simulink model "Koudruped_simcape"  (R2025b)
settings: Solver=VariableStepAuto  StartTime=0.0  StopTime=30  RelTol=1e-2
undefined symbols (not defined in the file or in its folder): fractalcoef, smiData, X, Y, Z
libraries: sm_lib x589, nesl_utility x93, slpidlib x5, mspsensorlib x4, simulink_extras x4, mspfiltlib x3, simulink x2
(part 16 of 16)

== matlab function Koudruped_simcape/Right Back Step2/MATLAB Function1 ==
  data: t input; pos output; phase_offset input; H_hedef input
function pos = fcn(t, phase_offset, H_hedef)
    pos = zeros(3,1); 
    
    % --- PARAMETRELER (Senin Orijinal Değerlerin) ---
    T_kalkis = 2.0;      
    T_bekleme = 1.0;     
    T_periyot = 1.0;     
    Duty_Factor = 0.5;   
    
    L_adim = 80;         
    H_adim = 30;         
    H_baslangic = -50;   
    Y_offset = 60;       
    
    % --- DURUM MAKİNESİ ---
    if t < T_kalkis
        z = H_baslangic + (H_hedef - H_baslangic) * (t / T_kalkis);
        x = 0;
        pos = [x; Y_offset; z];
        
    elseif t < (T_kalkis + T_bekleme)
        z = H_hedef;
        x = 0;
        pos = [x; Y_offset; z];
        
    else
        t_yurume = t - (T_kalkis + T_bekleme);
        
        T_fade = 2.0; 
        k_amp = min(t_yurume / T_fade, 1.0); 
        
        L_aktif = L_adim * k_amp;
        H_aktif = H_adim * k_amp;
        
        t_norm = mod((t_yurume / T_periyot) + phase_offset, 1.0);
        
        if t_norm < Duty_Factor
            % --- SWING PHASE (HAVADA İLERİ ATILMA) ---
            t_swing = t_norm / Duty_Factor; 
            
            x = (L_aktif/2) - L_aktif * (t_swing - sin(2*pi*t_swing)/(2*pi));
            z = H_hedef + H_aktif * sin(pi * t_swing); 
        else
            % --- STANCE PHASE (YERDE İTME) ---
            t_stance = (t_norm - Duty_Factor) / (1 - Duty_Factor);
            
            x_start = -(L_aktif/2);
            x_end = (L_aktif/2);
            x = x_start + (x_end - x_start) * ((1 - cos(pi * t_stance)) / 2);
            z = H_hedef;
        end
        
        pos = [x; Y_offset; z];
    end
end

== matlab function Koudruped_simcape/Right Back Step2/MATLAB Function2 ==
  data: pos input; angles output
function angles = inverse(pos)
    x = pos(1); y = pos(2); z = pos(3);
    
    % --- PARAMETRELER (Senin değerlerin) ---
    L1 = 44.41; a1 = 24.51; L2 = 100; L3 = 100;
    
    % --- 1. OMUZ (ROLL) ---
    theta1_rad = atan2(y, -z) - atan2(L1, sqrt(y^2 + z^2 - L1^2));

    % --- 2. YARDIMCI KOORDİNATLAR ---
    % Bacak düzlemindeki izdüşüm
    r = sqrt(y^2 + z^2 - L1^2) - a1;
    % Yeni düzlemde hedef noktası (x, r)
    dist_sq = x^2 + r^2;
    dist = sqrt(dist_sq);

    % --- 3. DİZ (KNEE) ---
    cos_phi = (L2^2 + L3^2 - dist_sq) / (2 * L2 * L3);
    cos_phi = min(max(cos_phi, -1), 1); % Sayısal koruma
    phi = acos(cos_phi);
    theta3_rad = (pi - phi); 

    % --- 4. KALÇA (PITCH) ---
    alpha = atan2(x, r);
cos_beta = (L2^2 + dist_sq - L3^2) / (2 * L2 * dist);
cos_beta = min(max(cos_beta, -1), 1);  % Sayısal koruma
beta = acos(cos_beta);
    theta2_rad = alpha + beta;

    % RAD -> DEG
    angles = [theta1_rad; theta2_rad; theta3_rad] * (180/pi);
end

== matlab function Koudruped_simcape/Right Front Step2/MATLAB Function12 ==
  data: t input; pos output; phase_offset input; H_hedef input
function pos = fcn(t, phase_offset, H_hedef)
    pos = zeros(3,1); 
    
    % --- PARAMETRELER  ---
    T_kalkis = 2.0;      
    T_bekleme = 1.0;     
    T_periyot = 1.0;     
    Duty_Factor = 0.5;   
    
    L_adim = 80;         
    H_adim = 30;         
    H_baslangic = -50;   
    Y_offset = 60;       
    
    % --- DURUM MAKİNESİ ---
    if t < T_kalkis
        z = H_baslangic + (H_hedef - H_baslangic) * (t / T_kalkis);
        x = 0;
        pos = [x; Y_offset; z];
        
    elseif t < (T_kalkis + T_bekleme)
        z = H_hedef;
        x = 0;
        pos = [x; Y_offset; z];
        
    else
        t_yurume = t - (T_kalkis + T_bekleme);
        
        T_fade = 2.0; 
        k_amp = min(t_yurume / T_fade, 1.0); 
        
        L_aktif = L_adim * k_amp;
        H_aktif = H_adim * k_amp;
        
        t_norm = mod((t_yurume / T_periyot) + phase_offset, 1.0);
        
        if t_norm < Duty_Factor
            % --- SWING PHASE (HAVADA İLERİ ATILMA) ---
            t_swing = t_norm / Duty_Factor; 
            
            x = (L_aktif/2) - L_aktif * (t_swing - sin(2*pi*t_swing)/(2*pi));
            z = H_hedef + H_aktif * sin(pi * t_swing); 
        else
            % --- STANCE PHASE (YERDE İTME) ---
            t_stance = (t_norm - Duty_Factor) / (1 - Duty_Factor);
            
            x_start = -(L_aktif/2);
            x_end = (L_aktif/2);
            x = x_start + (x_end - x_start) * ((1 - cos(pi * t_stance)) / 2);
            z = H_hedef;
        end
        
        pos = [x; Y_offset; z];
    end
end

== matlab function Koudruped_simcape/Right Front Step2/MATLAB Function13 ==
  data: pos input; angles output
function angles = inverse(pos)
    x = pos(1); y = pos(2); z = pos(3);
    
    % --- PARAMETRELER (Senin değerlerin) ---
    L1 = 44.41; a1 = 24.51; L2 = 100; L3 = 100;
    
    % --- 1. OMUZ (ROLL) ---
    theta1_rad = atan2(y, -z) - atan2(L1, sqrt(y^2 + z^2 - L1^2));

    % --- 2. YARDIMCI KOORDİNATLAR ---
    % Bacak düzlemindeki izdüşüm
    r = sqrt(y^2 + z^2 - L1^2) - a1;
    % Yeni düzlemde hedef noktası (x, r)
    dist_sq = x^2 + r^2;
    dist = sqrt(dist_sq);

    % --- 3. DİZ (KNEE) ---
    cos_phi = (L2^2 + L3^2 - dist_sq) / (2 * L2 * L3);
    cos_phi = min(max(cos_phi, -1), 1); % Sayısal koruma
    phi = acos(cos_phi);
    theta3_rad = (pi - phi); 

    % --- 4. KALÇA (PITCH) ---
    alpha = atan2(x, r);
cos_beta = (L2^2 + dist_sq - L3^2) / (2 * L2 * dist);
cos_beta = min(max(cos_beta, -1), 1);  % Sayısal koruma
beta = acos(cos_beta);
    theta2_rad = alpha + beta;

    % RAD -> DEG
    angles = [theta1_rad; theta2_rad; theta3_rad] * (180/pi);
end

== matlab function Koudruped_simcape/Left Back Step3/MATLAB Function1 ==
  data: t input; pos output; phase_offset input; H_hedef input
function pos = fcn(t, phase_offset, H_hedef)
    pos = zeros(3,1); 
    
    % --- PARAMETRELER (Senin Orijinal Değerlerin) ---
    T_kalkis = 2.0;      
    T_bekleme = 1.0;     
    T_periyot = 1.0;     
    Duty_Factor = 0.5;   
    
    L_adim = 80;         
    H_adim = 30;         
    H_baslangic = -50;   
    Y_offset = 60;       
    
    % --- DURUM MAKİNESİ ---
    if t < T_kalkis
        z = H_baslangic + (H_hedef - H_baslangic) * (t / T_kalkis);
        x = 0;
        pos = [x; Y_offset; z];
        
    elseif t < (T_kalkis + T_bekleme)
        z = H_hedef;
        x = 0;
        pos = [x; Y_offset; z];
        
    else
        t_yurume = t - (T_kalkis + T_bekleme);
        
        T_fade = 2.0; 
        k_amp = min(t_yurume / T_fade, 1.0); 
        
        L_aktif = L_adim * k_amp;
        H_aktif = H_adim * k_amp;
        
        t_norm = mod((t_yurume / T_periyot) + phase_offset, 1.0);
        
        if t_norm < Duty_Factor
            % --- SWING PHASE (HAVADA İLERİ ATILMA) ---
            t_swing = t_norm / Duty_Factor; 
            
            % DEĞİŞİKLİK: İşaretler ters çevrildi (+L/2'den -L/2'ye doğru atılacak)
            x = (L_aktif/2) - L_aktif * (t_swing - sin(2*pi*t_swing)/(2*pi));
            z = H_hedef + H_aktif * sin(pi * t_swing); 
        else
            % --- STANCE PHASE (YERDE İTME) ---
            t_stance = (t_norm - Duty_Factor) / (1 - Duty_Factor);
            
            % DEĞİŞİKLİK: Başlangıç ve bitiş noktaları yer değiştirdi (-L/2'den +L/2'ye itecek)
            x_start = -(L_aktif/2);
            x_end = (L_aktif/2);
            x = x_start + (x_end - x_start) * ((1 - cos(pi * t_stance)) / 2);
            z = H_hedef;
        end
        
        pos = [x; Y_offset; z];
    end
end

== matlab function Koudruped_simcape/Left Back Step3/MATLAB Function2 ==
  data: pos input; angles output
function angles = inverse(pos)
    x = pos(1); y = pos(2); z = pos(3);
    
    % --- PARAMETRELER (Senin değerlerin) ---
    L1 = 44.41; a1 = 24.51; L2 = 100; L3 = 100;
    
    % --- 1. OMUZ (ROLL) ---
    % Omuzun dışa doğru açılması için atan2 parametrelerini kontrol et
    % Eğer omuz içeri katlanıyorsa 'y' yerine '-y' deneyebilirsin
    theta1_rad = atan2(y, -z) - atan2(L1, sqrt(y^2 + z^2 - L1^2));

    % --- 2. YARDIMCI KOORDİNATLAR ---
    % Bacak düzlemindeki izdüşüm
    r = sqrt(y^2 + z^2 - L1^2) - a1;
    % Yeni düzlemde hedef noktası (x, r)
    dist_sq = x^2 + r^2;
    dist = sqrt(dist_sq);

    % --- 3. DİZ (KNEE) ---
    cos_phi = (L2^2 + L3^2 - dist_sq) / (2 * L2 * L3);
    cos_phi = min(max(cos_phi, -1), 1); % Sayısal koruma
    phi = acos(cos_phi);
    % theta3'ü pozitif yaparsan diz ters yöne kırılır
    theta3_rad = (pi - phi); 

    % --- 4. KALÇA (PITCH) ---
    alpha = atan2(x, r);
    beta = acos((L2^2 + dist_sq - L3^2) / (2 * L2 * dist));
    theta2_rad = alpha + beta;

    % RAD -> DEG
    angles = [theta1_rad; theta2_rad; theta3_rad] * (180/pi);
end

== matlab function Koudruped_simcape/Left Front Step/MATLAB Function2 ==
  data: pos input; angles output
function angles = inverse(pos)
    x = pos(1); y = pos(2); z = pos(3);
    
    % --- PARAMETRELER (Senin değerlerin) ---
    L1 = 44.41; a1 = 24.51; L2 = 100; L3 = 100;
    
    % --- 1. OMUZ (ROLL) ---
    theta1_rad = atan2(y, -z) - atan2(L1, sqrt(y^2 + z^2 - L1^2));

    % --- 2. YARDIMCI KOORDİNATLAR ---
    % Bacak düzlemindeki izdüşüm
    r = sqrt(y^2 + z^2 - L1^2) - a1;
    % Yeni düzlemde hedef noktası (x, r)
    dist_sq = x^2 + r^2;
    dist = sqrt(dist_sq);

    % --- 3. DİZ (KNEE) ---
    cos_phi = (L2^2 + L3^2 - dist_sq) / (2 * L2 * L3);
    cos_phi = min(max(cos_phi, -1), 1); % Sayısal koruma
    phi = acos(cos_phi);
    % theta3'ü pozitif yaparsan diz ters yöne kırılır
    theta3_rad = -(pi - phi); 

    % --- 4. KALÇA (PITCH) ---
    alpha = atan2(x, r);
    beta = acos((L2^2 + dist_sq - L3^2) / (2 * L2 * dist));
    theta2_rad = alpha + beta;

    % RAD -> DEG
    angles = [theta1_rad; theta2_rad; theta3_rad] * (180/pi);
end

== matlab function Koudruped_simcape/Left Front Step3/MATLAB Function1 ==
  data: t input; pos output; phase_offset input; H_hedef input
function pos = fcn(t, phase_offset, H_hedef)
    pos = zeros(3,1); 
    
    % --- PARAMETRELER (Senin Orijinal Değerlerin) ---
    T_kalkis = 2.0;      
    T_bekleme = 1.0;     
    T_periyot = 1.0;     
    Duty_Factor = 0.5;   
    
    L_adim = 80;         
    H_adim = 30;         
    H_baslangic = -50;   
    Y_offset = 60;       
    
    % --- DURUM MAKİNESİ ---
    if t < T_kalkis
        z = H_baslangic + (H_hedef - H_baslangic) * (t / T_kalkis);
        x = 0;
        pos = [x; Y_offset; z];
        
    elseif t < (T_kalkis + T_bekleme)
        z = H_hedef;
        x = 0;
        pos = [x; Y_offset; z];
        
    else
        t_yurume = t - (T_kalkis + T_bekleme);
        
        T_fade = 2.0; 
        k_amp = min(t_yurume / T_fade, 1.0); 
        
        L_aktif = L_adim * k_amp;
        H_aktif = H_adim * k_amp;
        
        t_norm = mod((t_yurume / T_periyot) + phase_offset, 1.0);
        
        if t_norm < Duty_Factor
            % --- SWING PHASE (HAVADA İLERİ ATILMA) ---
            t_swing = t_norm / Duty_Factor; 
            
            % DEĞİŞİKLİK: İşaretler ters çevrildi (+L/2'den -L/2'ye doğru atılacak)
            x = (L_aktif/2) - L_aktif * (t_swing - sin(2*pi*t_swing)/(2*pi));
            z = H_hedef + H_aktif * sin(pi * t_swing); 
        else
            % --- STANCE PHASE (YERDE İTME) ---
            t_stance = (t_norm - Duty_Factor) / (1 - Duty_Factor);
            
            % DEĞİŞİKLİK: Başlangıç ve bitiş noktaları yer değiştirdi (-L/2'den +L/2'ye itecek)
            x_start = -(L_aktif/2);
            x_end = (L_aktif/2);
            x = x_start + (x_end - x_start) * ((1 - cos(pi * t_stance)) / 2);
            z = H_hedef;
        end
        
        pos = [x; Y_offset; z];
    end
end

== matlab function Koudruped_simcape/Left Front Step3/MATLAB Function2 ==
  data: pos input; angles output
function angles = inverse(pos)
    x = pos(1); y = pos(2); z = pos(3);
    
    % --- PARAMETRELER (Senin değerlerin) ---
    L1 = 44.41; a1 = 24.51; L2 = 100; L3 = 100;
    
    % --- 1. OMUZ (ROLL) ---
    theta1_rad = atan2(y, -z) - atan2(L1, sqrt(y^2 + z^2 - L1^2));

    % --- 2. YARDIMCI KOORDİNATLAR ---
    % Bacak düzlemindeki izdüşüm
    r = sqrt(y^2 + z^2 - L1^2) - a1;
    % Yeni düzlemde hedef noktası (x, r)
    dist_sq = x^2 + r^2;
    dist = sqrt(dist_sq);

    % --- 3. DİZ (KNEE) ---
    cos_phi = (L2^2 + L3^2 - dist_sq) / (2 * L2 * L3);
    cos_phi = min(max(cos_phi, -1), 1); % Sayısal koruma
    phi = acos(cos_phi);
    % theta3'ü pozitif yaparsan diz ters yöne kırılır
    theta3_rad = (pi - phi); 

    % --- 4. KALÇA (PITCH) ---
    alpha = atan2(x, r);
    beta = acos((L2^2 + dist_sq - L3^2) / (2 * L2 * dist));
    theta2_rad = alpha + beta;

    % RAD -> DEG
    angles = [theta1_rad; theta2_rad; theta3_rad] * (180/pi);
end

== matlab function Koudruped_simcape/Right Back Step3/MATLAB Function1 ==
  data: t input; pos output; phase_offset input; H_hedef input
function pos = fcn(t, phase_offset, H_hedef)
    pos = zeros(3,1); 
    
    % --- PARAMETRELER (Senin Orijinal Değerlerin) ---
    T_kalkis = 2.0;      
    T_bekleme = 1.0;     
    T_periyot = 1.0;     
    Duty_Factor = 0.5;   
    
    L_adim = 80;         
    H_adim = 30;         
    H_baslangic = -50;   
    Y_offset = 60;       
    
    % --- DURUM MAKİNESİ ---
    if t < T_kalkis
        z = H_baslangic + (H_hedef - H_baslangic) * (t / T_kalkis);
        x = 0;
        pos = [x; Y_offset; z];
        
    elseif t < (T_kalkis + T_bekleme)
        z = H_hedef;
        x = 0;
        pos = [x; Y_offset; z];
        
    else
        t_yurume = t - (T_kalkis + T_bekleme);
        
        T_fade = 2.0; 
        k_amp = min(t_yurume / T_fade, 1.0); 
        
        L_aktif = L_adim * k_amp;
        H_aktif = H_adim * k_amp;
        
        t_norm = mod((t_yurume / T_periyot) + phase_offset, 1.0);
        
        if t_norm < Duty_Factor
            % --- SWING PHASE (HAVADA İLERİ ATILMA) ---
            t_swing = t_norm / Duty_Factor; 
            
            % DEĞİŞİKLİK: İşaretler ters çevrildi (+L/2'den -L/2'ye doğru atılacak)
            x = (L_aktif/2) - L_aktif * (t_swing - sin(2*pi*t_swing)/(2*pi));
            z = H_hedef + H_aktif * sin(pi * t_swing); 
        else
            % --- STANCE PHASE (YERDE İTME) ---
            t_stance = (t_norm - Duty_Factor) / (1 - Duty_Factor);
            
            % DEĞİŞİKLİK: Başlangıç ve bitiş noktaları yer değiştirdi (-L/2'den +L/2'ye itecek)
            x_start = -(L_aktif/2);
            x_end = (L_aktif/2);
            x = x_start + (x_end - x_start) * ((1 - cos(pi * t_stance)) / 2);
            z = H_hedef;
        end
        
        pos = [x; Y_offset; z];
    end
end

== matlab function Koudruped_simcape/Right Back Step3/MATLAB Function2 ==
  data: pos input; angles output
function angles = inverse(pos)
    x = pos(1); y = pos(2); z = pos(3);
    
    % --- PARAMETRELER (Senin değerlerin) ---
    L1 = 44.41; a1 = 24.51; L2 = 100; L3 = 100;
    
    % --- 1. OMUZ (ROLL) ---
    % Omuzun dışa doğru açılması için atan2 parametrelerini kontrol et
    % Eğer omuz içeri katlanıyorsa 'y' yerine '-y' deneyebilirsin
    theta1_rad = atan2(y, -z) - atan2(L1, sqrt(y^2 + z^2 - L1^2));

    % --- 2. YARDIMCI KOORDİNATLAR ---
    % Bacak düzlemindeki izdüşüm
    r = sqrt(y^2 + z^2 - L1^2) - a1;
    % Yeni düzlemde hedef noktası (x, r)
    dist_sq = x^2 + r^2;
    dist = sqrt(dist_sq);

    % --- 3. DİZ (KNEE) ---
    cos_phi = (L2^2 + L3^2 - dist_sq) / (2 * L2 * L3);
    cos_phi = min(max(cos_phi, -1), 1); % Sayısal koruma
    phi = acos(cos_phi);
    % theta3'ü pozitif yaparsan diz ters yöne kırılır
    theta3_rad = (pi - phi); 

    % --- 4. KALÇA (PITCH) ---
    alpha = atan2(x, r);
    beta = acos((L2^2 + dist_sq - L3^2) / (2 * L2 * dist));
    theta2_rad = alpha + beta;

    % RAD -> DEG
    angles = [theta1_rad; theta2_rad; theta3_rad] * (180/pi);
end

== matlab function Koudruped_simcape/Right Front Step3/MATLAB Function12 ==
  data: t input; pos output; phase_offset input; H_hedef input
function pos = fcn(t, phase_offset, H_hedef)
    pos = zeros(3,1); 
    
    % --- PARAMETRELER (Senin Orijinal Değerlerin) ---
    T_kalkis = 2.0;      
    T_bekleme = 1.0;     
    T_periyot = 1.0;     
    Duty_Factor = 0.5;   
    
    L_adim = 80;         
    H_adim = 30;         
    H_baslangic = -50;   
    Y_offset = 60;       
    
    % --- DURUM MAKİNESİ ---
    if t < T_kalkis
        z = H_baslangic + (H_hedef - H_baslangic) * (t / T_kalkis);
        x = 0;
        pos = [x; Y_offset; z];
        
    elseif t < (T_kalkis + T_bekleme)
        z = H_hedef;
        x = 0;
        pos = [x; Y_offset; z];
        
    else
        t_yurume = t - (T_kalkis + T_bekleme);
        
        T_fade = 2.0; 
        k_amp = min(t_yurume / T_fade, 1.0); 
        
        L_aktif = L_adim * k_amp;
        H_aktif = H_adim * k_amp;
        
        t_norm = mod((t_yurume / T_periyot) + phase_offset, 1.0);
        
        if t_norm < Duty_Factor
            % --- SWING PHASE (HAVADA İLERİ ATILMA) ---
            t_swing = t_norm / Duty_Factor; 
            
            % DEĞİŞİKLİK: İşaretler ters çevrildi (+L/2'den -L/2'ye doğru atılacak)
            x = (L_aktif/2) - L_aktif * (t_swing - sin(2*pi*t_swing)/(2*pi));
            z = H_hedef + H_aktif * sin(pi * t_swing); 
        else
            % --- STANCE PHASE (YERDE İTME) ---
            t_stance = (t_norm - Duty_Factor) / (1 - Duty_Factor);
            
            % DEĞİŞİKLİK: Başlangıç ve bitiş noktaları yer değiştirdi (-L/2'den +L/2'ye itecek)
            x_start = -(L_aktif/2);
            x_end = (L_aktif/2);
            x = x_start + (x_end - x_start) * ((1 - cos(pi * t_stance)) / 2);
            z = H_hedef;
        end
        
        pos = [x; Y_offset; z];
    end
end

== matlab function Koudruped_simcape/Right Front Step3/MATLAB Function13 ==
  data: pos input; angles output
function angles = inverse(pos)
    x = pos(1); y = pos(2); z = pos(3);
    
    % --- PARAMETRELER (Senin değerlerin) ---
    L1 = 44.41; a1 = 24.51; L2 = 100; L3 = 100;
    
    % --- 1. OMUZ (ROLL) ---
    % Omuzun dışa doğru açılması için atan2 parametrelerini kontrol et
    % Eğer omuz içeri katlanıyorsa 'y' yerine '-y' deneyebilirsin
    theta1_rad = atan2(y, -z) - atan2(L1, sqrt(y^2 + z^2 - L1^2));

    % --- 2. YARDIMCI KOORDİNATLAR ---
    % Bacak düzlemindeki izdüşüm
    r = sqrt(y^2 + z^2 - L1^2) - a1;
    % Yeni düzlemde hedef noktası (x, r)
    dist_sq = x^2 + r^2;
    dist = sqrt(dist_sq);

    % --- 3. DİZ (KNEE) ---
    cos_phi = (L2^2 + L3^2 - dist_sq) / (2 * L2 * L3);
    cos_phi = min(max(cos_phi, -1), 1); % Sayısal koruma
    phi = acos(cos_phi);
    % theta3'ü pozitif yaparsan diz ters yöne kırılır
    theta3_rad = (pi - phi); 

    % --- 4. KALÇA (PITCH) ---
    alpha = atan2(x, r);
    beta = acos((L2^2 + dist_sq - L3^2) / (2 * L2 * dist));
    theta2_rad = alpha + beta;

    % RAD -> DEG
    angles = [theta1_rad; theta2_rad; theta3_rad] * (180/pi);
end

== matlab function Koudruped_simcape/IMU2/MATLAB Function ==
  data: accel input; pitch_deg output
function pitch_deg = accelToPitch(accel)
%#codegen
    % Force input to be a 3-element vector
    accel_vec = zeros(3,1);
    accel_vec(1) = accel(1);
    accel_vec(2) = accel(2);
    accel_vec(3) = accel(3);
    
    ax = double(accel_vec(1));
    ay = double(accel_vec(2));
    az = double(accel_vec(3));
    
    pitch_rad = atan2(-az, ay);
    pitch_deg = pitch_rad * 180/pi;
end

== matlab function Koudruped_simcape/Left Back Step/MATLAB Function1 ==
  data: t input; pos output; phase_offset input; H_hedef input
function pos = fcn(t, phase_offset, H_hedef)
    pos = zeros(3,1); 
    
    % --- PARAMETRELER ---
    T_kalkis = 2.0;      
    T_bekleme = 1.0;     
    T_periyot = 1.0;     
    Duty_Factor = 0.5;   
    
    L_adim = 80;         
    H_adim = 30;         
    H_baslangic = -50;   
    Y_offset = 60;       
    
    % --- DURUM MAKİNESİ ---
    if t < T_kalkis
        z = H_baslangic + (H_hedef - H_baslangic) * (t / T_kalkis);
        x = 0;
        pos = [x; Y_offset; z];
        
    elseif t < (T_kalkis + T_bekleme)
        z = H_hedef;
        x = 0;
        pos = [x; Y_offset; z];
        
    else
        t_yurume = t - (T_kalkis + T_bekleme);
        
        % === FADE-IN (YUMUŞAK BAŞLANGIÇ) ÇARPANI ===
        % İlk 2 saniye boyunca adım boyu ve yüksekliği 0'dan 100%'e çıkar
        T_fade = 2.0; 
        k_amp = min(t_yurume / T_fade, 1.0); 
        
        % O anki aktif adım limitleri
        L_aktif = L_adim * k_amp;
        H_aktif = H_adim * k_amp;
        
        t_norm = mod((t_yurume / T_periyot) + phase_offset, 1.0);
        
        if t_norm < Duty_Factor
            % Swing Phase
            t_swing = t_norm / Duty_Factor; 
            x = -(L_aktif/2) + L_aktif * (t_swing - sin(2*pi*t_swing)/(2*pi));
            z = H_hedef + H_aktif * sin(pi * t_swing); 
        else
            % Stance Phase
            t_stance = (t_norm - Duty_Factor) / (1 - Duty_Factor);
            x_start = L_aktif/2;
            x_end = -(L_aktif/2);
            x = x_start + (x_end - x_start) * ((1 - cos(pi * t_stance)) / 2);
            z = H_hedef;
        end
        
        pos = [x; Y_offset; z];
    end
end

== matlab function Koudruped_simcape/Left Back Step/MATLAB Function2 ==
  data: pos input; angles output
function angles = inverse(pos)
    x = pos(1); y = pos(2); z = pos(3);
    
    % --- PARAMETRELER (Senin değerlerin) ---
    L1 = 44.41; a1 = 24.51; L2 = 100; L3 = 100;
    
    % --- 1. OMUZ (ROLL) ---
    % Omuzun dışa doğru açılması için atan2 parametrelerini kontrol et
    % Eğer omuz içeri katlanıyorsa 'y' yerine '-y' deneyebilirsin
    theta1_rad = atan2(y, -z) - atan2(L1, sqrt(y^2 + z^2 - L1^2));

    % --- 2. YARDIMCI KOORDİNATLAR ---
    % Bacak düzlemindeki izdüşüm
    r = sqrt(y^2 + z^2 - L1^2) - a1;
    % Yeni düzlemde hedef noktası (x, r)
    dist_sq = x^2 + r^2;
    dist = sqrt(dist_sq);

    % --- 3. DİZ (KNEE) ---
    cos_phi = (L2^2 + L3^2 - dist_sq) / (2 * L2 * L3);
    cos_phi = min(max(cos_phi, -1), 1); % Sayısal koruma
    phi = acos(cos_phi);
    % theta3'ü pozitif yaparsan diz ters yöne kırılır
    theta3_rad = -(pi - phi); 

    % --- 4. KALÇA (PITCH) ---
    alpha = atan2(x, r);
    beta = acos((L2^2 + dist_sq - L3^2) / (2 * L2 * dist));
    theta2_rad = alpha + beta;

    % RAD -> DEG
    angles = [theta1_rad; theta2_rad; theta3_rad] * (180/pi);
end

== matlab function Koudruped_simcape/Sağ Arka Adım1/MATLAB Function1 ==
  data: t input; pos output; phase_offset input
function pos = fcn(t, phase_offset)
    pos = zeros(3,1); 
    
    % --- PARAMETRELER ---
    T_kalkis = 2.0;      
    T_bekleme = 1.0;     
    T_periyot = 2.0;     % Walk gait daha yavaştır, stabilite için 1.0'dan 2.0'a çıkarıldı.
    Swing_Ratio = 0.25;  % Walk gait için havada kalma süresi periyodun %25'i olmalı.
    
    L_adim = 80;         
    H_adim = 30;         
    H_baslangic = -50;   
    H_hedef = -130;
    Y_offset = 60;       
    
    % --- DURUM MAKİNESİ ---
    if t < T_kalkis
        z = H_baslangic + (H_hedef - H_baslangic) * (t / T_kalkis);
        x = 0;
        pos = [x; Y_offset; z];
        
    elseif t < (T_kalkis + T_bekleme)
        z = H_hedef-2;
        x = 0;
        pos = [x; Y_offset; z];
        
    else
        t_yurume = t - (T_kalkis + T_bekleme);
        
        % === FADE-IN (YUMUŞAK BAŞLANGIÇ) ÇARPANI ===
        T_fade = 2.0; 
        k_amp = min(t_yurume / T_fade, 1.0); 
        
        L_aktif = L_adim * k_amp;
        H_aktif = H_adim * k_amp;
        
        t_norm = mod((t_yurume / T_periyot) + phase_offset, 1.0);
        
        if t_norm < Swing_Ratio
            % Swing Phase (Havada)
            t_swing = t_norm / Swing_Ratio; 
            x = -(L_aktif/2) + L_aktif * (t_swing - sin(2*pi*t_swing)/(2*pi));
            z = H_hedef + H_aktif * sin(pi * t_swing); 
        else
            % Stance Phase (Yerde İtme)
            t_stance = (t_norm - Swing_Ratio) / (1 - Swing_Ratio);
            x_start = L_aktif/2;
            x_end = -(L_aktif/2);
            x = x_start + (x_end - x_start) * ((1 - cos(pi * t_stance)) / 2);
            z = H_hedef;
        end
        
        pos = [x; Y_offset; z];
    end
end

== matlab function Koudruped_simcape/Sağ Arka Adım1/MATLAB Function2 ==
  data: pos input; angles output
function angles = inverse(pos)
    x = pos(1); y = pos(2); z = pos(3);
    
    % --- PARAMETRELER (Senin değerlerin) ---
    L1 = 44.41; a1 = 24.51; L2 = 100; L3 = 102.5;
    
    % --- 1. OMUZ (ROLL) ---
    % Omuzun dışa doğru açılması için atan2 parametrelerini kontrol et
    % Eğer omuz içeri katlanıyorsa 'y' yerine '-y' deneyebilirsin
    theta1_rad = atan2(y, -z) - atan2(L1, sqrt(y^2 + z^2 - L1^2));

    % --- 2. YARDIMCI KOORDİNATLAR ---
    % Bacak düzlemindeki izdüşüm
    r = sqrt(y^2 + z^2 - L1^2) - a1;
    % Yeni düzlemde hedef noktası (x, r)
    dist_sq = x^2 + r^2;
    dist = sqrt(dist_sq);

    % --- 3. DİZ (KNEE) ---
    cos_phi = (L2^2 + L3^2 - dist_sq) / (2 * L2 * L3);
    cos_phi = min(max(cos_phi, -1), 1); % Sayısal koruma
    phi = acos(cos_phi);
    % theta3'ü pozitif yaparsan diz ters yöne kırılır
    theta3_rad = -(pi - phi); 

    % --- 4. KALÇA (PITCH) ---
    alpha = atan2(x, r);
    beta = acos((L2^2 + dist_sq - L3^2) / (2 * L2 * dist));
    theta2_rad = alpha + beta;

    % RAD -> DEG
    angles = [theta1_rad; theta2_rad; theta3_rad] * (180/pi);
end

== matlab function Koudruped_simcape/Sağ Ön Adım1/MATLAB Function12 ==
  data: t input; pos output; phase_offset input
function pos = fcn(t, phase_offset)
    pos = zeros(3,1); 
    
    % --- PARAMETRELER ---
    T_kalkis = 2.0;      
    T_bekleme = 1.0;     
    T_periyot = 2.0;     % Walk gait daha yavaştır, stabilite için 1.0'dan 2.0'a çıkarıldı.
    Swing_Ratio = 0.25;  % Walk gait için havada kalma süresi periyodun %25'i olmalı.
    
    L_adim = 80;         
    H_adim = 30;         
    H_baslangic = -50;   
    H_hedef = -130;
    Y_offset = 60;       
    
    % --- DURUM MAKİNESİ ---
    if t < T_kalkis
        z = H_baslangic + (H_hedef - H_baslangic) * (t / T_kalkis);
        x = 0;
        pos = [x; Y_offset; z];
        
    elseif t < (T_kalkis + T_bekleme)
        z = H_hedef-2;
        x = 0;
        pos = [x; Y_offset; z];
        
    else
        t_yurume = t - (T_kalkis + T_bekleme);
        
        % === FADE-IN (YUMUŞAK BAŞLANGIÇ) ÇARPANI ===
        T_fade = 2.0; 
        k_amp = min(t_yurume / T_fade, 1.0); 
        
        L_aktif = L_adim * k_amp;
        H_aktif = H_adim * k_amp;
        
        t_norm = mod((t_yurume / T_periyot) + phase_offset, 1.0);
        
        if t_norm < Swing_Ratio
            % Swing Phase (Havada)
            t_swing = t_norm / Swing_Ratio; 
            x = -(L_aktif/2) + L_aktif * (t_swing - sin(2*pi*t_swing)/(2*pi));
            z = H_hedef + H_aktif * sin(pi * t_swing); 
        else
            % Stance Phase (Yerde İtme)
            t_stance = (t_norm - Swing_Ratio) / (1 - Swing_Ratio);
            x_start = L_aktif/2;
            x_end = -(L_aktif/2);
            x = x_start + (x_end - x_start) * ((1 - cos(pi * t_stance)) / 2);
            z = H_hedef;
        end
        
        pos = [x; Y_offset; z];
    end
end

== matlab function Koudruped_simcape/Sağ Ön Adım1/MATLAB Function13 ==
  data: pos input; angles output
function angles = inverse(pos)
    x = pos(1); y = pos(2); z = pos(3);
    
    % --- PARAMETRELER (Senin değerlerin) ---
    L1 = 44.41; a1 = 24.51; L2 = 100; L3 = 102.5;
    
    % --- 1. OMUZ (ROLL) ---
    % Omuzun dışa doğru açılması için atan2 parametrelerini kontrol et
    % Eğer omuz içeri katlanıyorsa 'y' yerine '-y' deneyebilirsin
    theta1_rad = atan2(y, -z) - atan2(L1, sqrt(y^2 + z^2 - L1^2));

    % --- 2. YARDIMCI KOORDİNATLAR ---
    % Bacak düzlemindeki izdüşüm
    r = sqrt(y^2 + z^2 - L1^2) - a1;
    % Yeni düzlemde hedef noktası (x, r)
    dist_sq = x^2 + r^2;
    dist = sqrt(dist_sq);

    % --- 3. DİZ (KNEE) ---
    cos_phi = (L2^2 + L3^2 - dist_sq) / (2 * L2 * L3);
    cos_phi = min(max(cos_phi, -1), 1); % Sayısal koruma
    phi = acos(cos_phi);
    % theta3'ü pozitif yaparsan diz ters yöne kırılır
    theta3_rad = -(pi - phi); 

    % --- 4. KALÇA (PITCH) ---
    alpha = atan2(x, r);
    beta = acos((L2^2 + dist_sq - L3^2) / (2 * L2 * dist));
    theta2_rad = alpha + beta;

    % RAD -> DEG
    angles = [theta1_rad; theta2_rad; theta3_rad] * (180/pi);
end

== matlab function Koudruped_simcape/Sol Arka Adım1/MATLAB Function1 ==
  data: t input; pos output; phase_offset input
function pos = fcn(t, phase_offset)
    pos = zeros(3,1); 
    
    % --- PARAMETRELER ---
    T_kalkis = 2.0;      
    T_bekleme = 1.0;     
    T_periyot = 2.0;     % Walk gait daha yavaştır, stabilite için 1.0'dan 2.0'a çıkarıldı.
    Swing_Ratio = 0.25;  % Walk gait için havada kalma süresi periyodun %25'i olmalı.
    
    L_adim = 80;         
    H_adim = 30;         
    H_baslangic = -50;   
    H_hedef = -130;
    Y_offset = 60;       
    
    % --- DURUM MAKİNESİ ---
    if t < T_kalkis
        z = H_baslangic + (H_hedef - H_baslangic) * (t / T_kalkis);
        x = 0;
        pos = [x; Y_offset; z];
        
    elseif t < (T_kalkis + T_bekleme)
        z = H_hedef-2;
        x = 0;
        pos = [x; Y_offset; z];
        
    else
        t_yurume = t - (T_kalkis + T_bekleme);
        
        % === FADE-IN (YUMUŞAK BAŞLANGIÇ) ÇARPANI ===
        T_fade = 2.0; 
        k_amp = min(t_yurume / T_fade, 1.0); 
        
        L_aktif = L_adim * k_amp;
        H_aktif = H_adim * k_amp;
        
        t_norm = mod((t_yurume / T_periyot) + phase_offset, 1.0);
        
        if t_norm < Swing_Ratio
            % Swing Phase (Havada)
            t_swing = t_norm / Swing_Ratio; 
            x = -(L_aktif/2) + L_aktif * (t_swing - sin(2*pi*t_swing)/(2*pi));
            z = H_hedef + H_aktif * sin(pi * t_swing); 
        else
            % Stance Phase (Yerde İtme)
            t_stance = (t_norm - Swing_Ratio) / (1 - Swing_Ratio);
            x_start = L_aktif/2;
            x_end = -(L_aktif/2);
            x = x_start + (x_end - x_start) * ((1 - cos(pi * t_stance)) / 2);
            z = H_hedef;
        end
        
        pos = [x; Y_offset; z];
    end
end

== matlab function Koudruped_simcape/Right Back Step/MATLAB Function1 ==
  data: t input; pos output; phase_offset input; H_hedef input
function pos = fcn(t, phase_offset, H_hedef)
    pos = zeros(3,1); 
    
    % --- PARAMETRELER ---
    T_kalkis = 2.0;      
    T_bekleme = 1.0;     
    T_periyot = 1.0;     
    Duty_Factor = 0.5;   
    
    L_adim = 80;         
    H_adim = 30;         
    H_baslangic = -50;   
    Y_offset = 60;       
    
    % --- DURUM MAKİNESİ ---
    if t < T_kalkis
        z = H_baslangic + (H_hedef - H_baslangic) * (t / T_kalkis);
        x = 0;
        pos = [x; Y_offset; z];
        
    elseif t < (T_kalkis + T_bekleme)
        z = H_hedef;
        x = 0;
        pos = [x; Y_offset; z];
        
    else
        t_yurume = t - (T_kalkis + T_bekleme);
        
        % === FADE-IN (YUMUŞAK BAŞLANGIÇ) ÇARPANI ===
        % İlk 2 saniye boyunca adım boyu ve yüksekliği 0'dan 100%'e çıkar
        T_fade = 2.0; 
        k_amp = min(t_yurume / T_fade, 1.0); 
        
        % O anki aktif adım limitleri
        L_aktif = L_adim * k_amp;
        H_aktif = H_adim * k_amp;
        
        t_norm = mod((t_yurume / T_periyot) + phase_offset, 1.0);
        
        if t_norm < Duty_Factor
            % Swing Phase
            t_swing = t_norm / Duty_Factor; 
            x = -(L_aktif/2) + L_aktif * (t_swing - sin(2*pi*t_swing)/(2*pi));
            z = H_hedef + H_aktif * sin(pi * t_swing); 
        else
            % Stance Phase
            t_stance = (t_norm - Duty_Factor) / (1 - Duty_Factor);
            x_start = L_aktif/2;
            x_end = -(L_aktif/2);
            x = x_start + (x_end - x_start) * ((1 - cos(pi * t_stance)) / 2);
            z = H_hedef;
        end
        
        pos = [x; Y_offset; z];
    end
end

== matlab function Koudruped_simcape/Sol Arka Adım1/MATLAB Function2 ==
  data: pos input; angles output
function angles = inverse(pos)
    x = pos(1); y = pos(2); z = pos(3);
    
    % --- PARAMETRELER (Senin değerlerin) ---
    L1 = 44.41; a1 = 24.51; L2 = 100; L3 = 102.5;
    
    % --- 1. OMUZ (ROLL) ---
    % Omuzun dışa doğru açılması için atan2 parametrelerini kontrol et
    % Eğer omuz içeri katlanıyorsa 'y' yerine '-y' deneyebilirsin
    theta1_rad = atan2(y, -z) - atan2(L1, sqrt(y^2 + z^2 - L1^2));

    % --- 2. YARDIMCI KOORDİNATLAR ---
    % Bacak düzlemindeki izdüşüm
    r = sqrt(y^2 + z^2 - L1^2) - a1;
    % Yeni düzlemde hedef noktası (x, r)
    dist_sq = x^2 + r^2;
    dist = sqrt(dist_sq);

    % --- 3. DİZ (KNEE) ---
    cos_phi = (L2^2 + L3^2 - dist_sq) / (2 * L2 * L3);
    cos_phi = min(max(cos_phi, -1), 1); % Sayısal koruma
    phi = acos(cos_phi);
    % theta3'ü pozitif yaparsan diz ters yöne kırılır
    theta3_rad = -(pi - phi); 

    % --- 4. KALÇA (PITCH) ---
    alpha = atan2(x, r);
    beta = acos((L2^2 + dist_sq - L3^2) / (2 * L2 * dist));
    theta2_rad = alpha + beta;

    % RAD -> DEG
    angles = [theta1_rad; theta2_rad; theta3_rad] * (180/pi);
end
